simulink model "s_b4a4x32kf_26"  (R2018a)
settings: Solver=VariableStepDiscrete  StartTime=0.0  StopTime=10000  RelTol=1e-3
undefined symbols (not defined in the file): fft_stages, n_bits_ants, n_bits_xengs
libraries: xbsIndex_r4 x21247, casper_library_misc x37, casper_library_scopes x13, casper_library_delays x8, xbsReplacements_r4 x6, xps_library x4
(part 36 of 268)

== system s_b4a4x32kf_26/sys1/xeng_pack_out ==
  note: if we become misaligned,
      | then we must flush the buffers
      | by reading one word, waiting "fifo_latency" clocks,
      | then reading another word until we get rb_done.
  note: the last packet
      | might be shorter!
  note: Delay the output from x-engines,
      | so that only one sends at a time.
  note: we must create a gap
      | between packets from
      | mutliple x-engines to allow
      | the buffers on the output switch
      | ports to drain and NIC card
      | to service the packets.
  data_in : Inport
  valid_in : Inport  Port=2
  pkt_rdy : Inport  Port=3
  rb_done : Inport  Port=4
  timestamp : Inport  Port=5
  xeng_id : Inport  Port=6
  go : Inport  Port=7
  gap_size : Inport  Port=8
  start_offset : Inport  Port=9
  AddSub1 : xbsIndex_r4/AddSub  mode=Subtraction  use_carryin=off  use_carryout=off  en=off  latency=1  precision=User Defined  arith_type=Unsigned  n_bits=vector_bits+1  bin_pt=0  quantization=Truncate  overflow=Saturate  use_behavioral_HDL=on  hw_selection=Fabric  pipelined=off  dbl_ovrd=off  block_type=addsub
      settings: SourceProductName=The database /home/jmanley/.matlab/R2018a/slblocks_master.db is locked, or a table in the database is locked. (database is locked)
  Concat : xbsIndex_r4/Concat  num_inputs=2  dbl_ovrd=off  block_type=concat
      settings: SourceProductName=The database /home/jmanley/.matlab/R2018a/slblocks_master.db is locked, or a table in the database is locked. (database is locked)
  Constant1 : xbsIndex_r4/Constant  const=0  gui_display_data_type=Fixed-point  arith_type=Unsigned  n_bits=spead_lsw  bin_pt=0  preci_type=Single  exp_width=8  frac_width=24  explicit_period=on  period=1  equ=P=C  opselect=C  inp2=PCIN>>17  opr=+  inp1=P  carry=CIN  dbl_ovrd=off  block_type=constant
      settings: SourceProductName=The database /home/jmanley/.matlab/R2018a/slblocks_master.db is locked, or a table in the database is locked. (database is locked)
  Constant15 : xbsIndex_r4/Constant  const=pkt_len  gui_display_data_type=Fixed-point  arith_type=Unsigned  n_bits=vector_bits+1  bin_pt=0  preci_type=Single  exp_width=8  frac_width=24  explicit_period=on  period=1  equ=P=C  opselect=C  inp2=PCIN>>17  opr=+  inp1=P  carry=CIN  dbl_ovrd=off  block_type=constant
      settings: SourceProductName=The database /home/jmanley/.matlab/R2018a/slblocks_master.db is locked, or a table in the database is locked. (database is locked)
  Constant2 : xbsIndex_r4/Constant  const=(vector_len)-1  gui_display_data_type=Fixed-point  arith_type=Unsigned  n_bits=vector_bits+1  bin_pt=0  preci_type=Single  exp_width=8  frac_width=24  explicit_period=on  period=1  equ=P=C  opselect=C  inp2=PCIN>>17  opr=+  inp1=P  carry=CIN  dbl_ovrd=off  block_type=constant
      settings: SourceProductName=The database /home/jmanley/.matlab/R2018a/slblocks_master.db is locked, or a table in the database is locked. (database is locked)
  Constant3 : xbsIndex_r4/Constant  const=vector_len  gui_display_data_type=Fixed-point  arith_type=Unsigned  n_bits=vector_bits+1  bin_pt=0  preci_type=Single  exp_width=8  frac_width=24  explicit_period=on  period=1  equ=P=C  opselect=C  inp2=PCIN>>17  opr=+  inp1=P  carry=CIN  dbl_ovrd=off  block_type=constant
      settings: SourceProductName=The database /home/jmanley/.matlab/R2018a/slblocks_master.db is locked, or a table in the database is locked. (database is locked)
  Constant6 : xbsIndex_r4/Constant  const=heap_len  gui_display_data_type=Fixed-point  arith_type=Unsigned  n_bits=spead_lsw  bin_pt=0  preci_type=Single  exp_width=8  frac_width=24  explicit_period=on  period=1  equ=P=C  opselect=C  inp2=PCIN>>17  opr=+  inp1=P  carry=CIN  dbl_ovrd=off  block_type=constant
      settings: SourceProductName=The database /home/jmanley/.matlab/R2018a/slblocks_master.db is locked, or a table in the database is locked. (database is locked)
  Constant7 : xbsIndex_r4/Constant  const=pkt_len-1  gui_display_data_type=Fixed-point  arith_type=Unsigned  n_bits=pkt_bits  bin_pt=0  preci_type=Single  exp_width=8  frac_width=24  explicit_period=on  period=1  equ=P=C  opselect=C  inp2=PCIN>>17  opr=+  inp1=P  carry=CIN  dbl_ovrd=off  block_type=constant
      settings: SourceProductName=The database /home/jmanley/.matlab/R2018a/slblocks_master.db is locked, or a table in the database is locked. (database is locked)
  Constant8 : xbsIndex_r4/Constant  const=1  gui_display_data_type=Fixed-point  arith_type=Unsigned  n_bits=ceil(log2(fifo_latency))+1  bin_pt=0  preci_type=Single  exp_width=8  frac_width=24  explicit_period=on  period=1  equ=P=C  opselect=C  inp2=PCIN>>17  opr=+  inp1=P  carry=CIN  dbl_ovrd=off  block_type=constant
      settings: SourceProductName=The database /home/jmanley/.matlab/R2018a/slblocks_master.db is locked, or a table in the database is locked. (database is locked)
  Convert{,1..4,6} (6 alike) : xbsIndex_r4/Convert  gui_display_data_type=Fixed-point  arith_type=Unsigned  n_bits=spead_lsw  bin_pt=0  float_type=Single  exp_bits=8  fraction_bits=24  quantization=Truncate  overflow=Wrap  en=off  latency=0  pipeline=off  dbl_ovrd=off  block_type=convert
      settings: SourceProductName=The database /home/jmanley/.matlab/R2018a/slblocks_master.db is locked, or a table in the database is locked. (database is locked)  block_version=11.4
  Counter1 : xbsIndex_r4/Counter  cnt_type=Free Running  cnt_to=1023  operation=Up  start_count=0  cnt_by_val=1  arith_type=Unsigned  n_bits=vector_bits+1  bin_pt=0  load_pin=off  rst=on  en=on  explicit_period=on  period=1  use_behavioral_HDL=off  implementation=Fabric  use_rpm=on  dbl_ovrd=off  block_type=counter
      settings: SourceProductName=The database /home/jmanley/.matlab/R2018a/slblocks_master.db is locked, or a table in the database is locked. (database is locked)  xl_area=[0, 0, 0, 0, 0, 0, 0]
  Delay{,3,10..17,24} (11 alike) : xbsIndex_r4/Delay  rst=off  infoeditControl=Selection of Reset will increase slice count due to use of real FFs and instead of SRLs  en=off  latency=1  reg_retiming=on  dbl_ovrd=off  block_type=delay
      settings: SourceProductName=The database /home/jmanley/.matlab/R2018a/slblocks_master.db is locked, or a table in the database is locked. (database is locked)  block_version=11.4
  Delay1 : xbsIndex_r4/Delay  rst=off  infoeditControl=Selection of Reset will increase slice count due to use of real FFs and instead of SRLs  en=on  latency=1  reg_retiming=on  dbl_ovrd=off  block_type=delay
      settings: SourceProductName=The database /home/jmanley/.matlab/R2018a/slblocks_master.db is locked, or a table in the database is locked. (database is locked)
  Delay2 : xbsIndex_r4/Delay  rst=off  infoeditControl=Selection of Reset will increase slice count due to use of real FFs and instead of SRLs  en=off  latency=fifo_latency  reg_retiming=on  dbl_ovrd=off  block_type=delay
      settings: SourceProductName=The database /home/jmanley/.matlab/R2018a/slblocks_master.db is locked, or a table in the database is locked. (database is locked)  block_version=11.4
  Delay4 : xbsIndex_r4/Delay  rst=off  infoeditControl=Selection of Reset will increase slice count due to use of real FFs and instead of SRLs  en=off  latency=fifo_latency  reg_retiming=on  dbl_ovrd=off  block_type=delay
      settings: SourceProductName=The database /home/jmanley/.matlab/R2018a/slblocks_master.db is locked, or a table in the database is locked. (database is locked)  block_version=11.4
  Delay5 : xbsIndex_r4/Delay  rst=off  infoeditControl=Selection of Reset will increase slice count due to use of real FFs and instead of SRLs  en=on  latency=1  reg_retiming=on  dbl_ovrd=off  block_type=delay
      settings: SourceProductName=The database /home/jmanley/.matlab/R2018a/slblocks_master.db is locked, or a table in the database is locked. (database is locked)
  Delay7 : xbsIndex_r4/Delay  rst=on  infoeditControl=Selection of Reset will increase slice count due to use of real FFs and instead of SRLs  en=on  latency=1  reg_retiming=on  dbl_ovrd=off  block_type=delay
      settings: SourceProductName=The database /home/jmanley/.matlab/R2018a/slblocks_master.db is locked, or a table in the database is locked. (database is locked)
  Delay8 : xbsIndex_r4/Delay  rst=on  infoeditControl=Selection of Reset will increase slice count due to use of real FFs and instead of SRLs  en=on  latency=1  reg_retiming=on  dbl_ovrd=off  block_type=delay
      settings: SourceProductName=The database /home/jmanley/.matlab/R2018a/slblocks_master.db is locked, or a table in the database is locked. (database is locked)
  Delay9 : xbsIndex_r4/Delay  rst=on  infoeditControl=Selection of Reset will increase slice count due to use of real FFs and instead of SRLs  en=on  latency=1  reg_retiming=on  dbl_ovrd=off  block_type=delay
      settings: SourceProductName=The database /home/jmanley/.matlab/R2018a/slblocks_master.db is locked, or a table in the database is locked. (database is locked)
  Inverter{1..3,6..7} (5 alike) : xbsIndex_r4/Inverter  en=off  latency=0  dbl_ovrd=off  block_type=inv
      settings: SourceProductName=The database /home/jmanley/.matlab/R2018a/slblocks_master.db is locked, or a table in the database is locked. (database is locked)  block_version=11.4
  Logical{1,3..5,13..14} (6 alike) : xbsIndex_r4/Logical  logical_function=OR  inputs=2  en=off  latency=0  precision=Full  arith_type=Unsigned  n_bits=8  bin_pt=2  align_bp=on  dbl_ovrd=off  block_type=logical
      settings: SourceProductName=The database /home/jmanley/.matlab/R2018a/slblocks_master.db is locked, or a table in the database is locked. (database is locked)  xl_area=[0, 0, 0, 0, 0, 0, 0]
  Logical{2,8..12,15} (7 alike) : xbsIndex_r4/Logical  logical_function=AND  inputs=2  en=off  latency=0  precision=Full  arith_type=Unsigned  n_bits=8  bin_pt=2  align_bp=on  dbl_ovrd=off  block_type=logical
      settings: SourceProductName=The database /home/jmanley/.matlab/R2018a/slblocks_master.db is locked, or a table in the database is locked. (database is locked)  xl_area=[0, 0, 0, 0, 0, 0, 0]
  Logical17 : xbsIndex_r4/Logical  logical_function=AND  inputs=2  en=off  latency=1  precision=Full  arith_type=Unsigned  n_bits=8  bin_pt=2  align_bp=on  dbl_ovrd=off  block_type=logical
      settings: SourceProductName=The database /home/jmanley/.matlab/R2018a/slblocks_master.db is locked, or a table in the database is locked. (database is locked)  xl_area=[0, 0, 0, 0, 0, 0, 0]
  Logical18 : xbsIndex_r4/Logical  logical_function=AND  inputs=2  en=off  latency=1  precision=Full  arith_type=Unsigned  n_bits=8  bin_pt=2  align_bp=on  dbl_ovrd=off  block_type=logical
      settings: SourceProductName=The database /home/jmanley/.matlab/R2018a/slblocks_master.db is locked, or a table in the database is locked. (database is locked)  xl_area=[0, 0, 0, 0, 0, 0, 0]
  Logical19 : xbsIndex_r4/Logical  logical_function=AND  inputs=2  en=off  latency=1  precision=Full  arith_type=Unsigned  n_bits=8  bin_pt=2  align_bp=on  dbl_ovrd=off  block_type=logical
      settings: SourceProductName=The database /home/jmanley/.matlab/R2018a/slblocks_master.db is locked, or a table in the database is locked. (database is locked)  xl_area=[0, 0, 0, 0, 0, 0, 0]
  Logical7 : xbsIndex_r4/Logical  logical_function=XOR  inputs=2  en=off  latency=0  precision=Full  arith_type=Unsigned  n_bits=8  bin_pt=2  align_bp=on  dbl_ovrd=off  block_type=logical
      settings: SourceProductName=The database /home/jmanley/.matlab/R2018a/slblocks_master.db is locked, or a table in the database is locked. (database is locked)  xl_area=[0, 0, 0, 0, 0, 0, 0]
  Mux1 : xbsIndex_r4/Mux  inputs=2  en=off  latency=1  precision=Full  arith_type="Signed  (2's comp)"  n_bits=8  bin_pt=2  quantization=Truncate  overflow=Wrap  dbl_ovrd=off  block_type=mux
      settings: SourceProductName=The database /home/jmanley/.matlab/R2018a/slblocks_master.db is locked, or a table in the database is locked. (database is locked)  xl_area=[0, 0, 0, 0, 0, 0, 0]
  Reinterpret : xbsIndex_r4/Reinterpret  force_arith_type=on  arith_type=Unsigned  force_bin_pt=on  bin_pt=0  block_type=reinterpret
      settings: SourceProductName=The database /home/jmanley/.matlab/R2018a/slblocks_master.db is locked, or a table in the database is locked. (database is locked)  infoedit="Changes signal type without altering the binary representation.   You can changed the signal between signed and unsigned, and relocate the binary point.<br><br>Hardware notes: In hardware this block costs nothing.<br><br>Example:  Suppose the input is 6 bits wide, signed, with 2 fractional bits, and the output is forced to unsigned with 0 fractional bits.  Then an input of -2.0 (1110.00 in binary 2's complement) becomes an output of 56 (111000 in binary)."
  Relational1 : xbsIndex_r4/Relational  mode=a=b  op_type=Bool  en=off  latency=0  dbl_ovrd=off  block_type=relational
      settings: SourceProductName=The database /home/jmanley/.matlab/R2018a/slblocks_master.db is locked, or a table in the database is locked. (database is locked)  xl_area=[0, 0, 0, 0, 0, 0, 0]  block_version=10.1.3
  Relational2 : xbsIndex_r4/Relational  mode=a<b  op_type=Bool  en=off  latency=0  dbl_ovrd=off  block_type=relational
      settings: SourceProductName=The database /home/jmanley/.matlab/R2018a/slblocks_master.db is locked, or a table in the database is locked. (database is locked)  xl_area=[0, 0, 0, 0, 0, 0, 0]  block_version=10.1.3
  Relational4 : xbsIndex_r4/Relational  mode=a=b  op_type=Bool  en=off  latency=0  dbl_ovrd=off  block_type=relational
      settings: SourceProductName=The database /home/jmanley/.matlab/R2018a/slblocks_master.db is locked, or a table in the database is locked. (database is locked)  xl_area=[0, 0, 0, 0, 0, 0, 0]  block_version=10.1.3
  Relational5 : xbsIndex_r4/Relational  mode=a=b  op_type=Bool  en=off  latency=0  dbl_ovrd=off  block_type=relational
      settings: SourceProductName=The database /home/jmanley/.matlab/R2018a/slblocks_master.db is locked, or a table in the database is locked. (database is locked)  xl_area=[0, 0, 0, 0, 0, 0, 0]  block_version=10.1.3
  Shift1 : xbsIndex_r4/Shift  shift_dir=Left  shift_bits=n_bits_word_size  en=off  latency=0  precision=Full  arith_type="Signed  (2's comp)"  n_bits=16  bin_pt=14  quantization=Truncate  overflow=Wrap  dbl_ovrd=off  block_type=shift
      settings: SourceProductName=The database /home/jmanley/.matlab/R2018a/slblocks_master.db is locked, or a table in the database is locked. (database is locked)
  Shift2 : xbsIndex_r4/Shift  shift_dir=Left  shift_bits=n_bits_chans  en=off  latency=0  precision=Full  arith_type="Signed  (2's comp)"  n_bits=16  bin_pt=14  quantization=Truncate  overflow=Wrap  dbl_ovrd=off  block_type=shift
      settings: SourceProductName=The database /home/jmanley/.matlab/R2018a/slblocks_master.db is locked, or a table in the database is locked. (database is locked)
  Slice : xbsIndex_r4/Slice  nbits=pkt_bits  boolean_output=off  mode=Lower Bit Location + Width  bit1=0  base1=MSB of Input  bit0=0  base0=LSB of Input  dbl_ovrd=off  block_type=slice
      settings: SourceProductName=The database /home/jmanley/.matlab/R2018a/slblocks_master.db is locked, or a table in the database is locked. (database is locked)
  Slice1 : xbsIndex_r4/Slice  nbits=1  boolean_output=off  mode=Two Bit Locations  bit1=0  base1=MSB of Input  bit0=n_bits_timestamp_padding  base0=LSB of Input  dbl_ovrd=off  block_type=slice
      settings: SourceProductName=The database /home/jmanley/.matlab/R2018a/slblocks_master.db is locked, or a table in the database is locked. (database is locked)
  edge_detect : Subsystem  AncestorBlock=casper_library_misc/edge_detect  mask(edge_detect){edge=Rising, polarity=Active High, x_in=[0 0.08 0.08 0.16 0.16 0.24 0.24 0.32 0.32 0.4], y_in=[-1 -1  1  1  1  1  1  1  1  1], x_out=[0.6 0.68 0.68 0.76 0.76 0.84 0.84 0.92 0.92 1], y_out=[-1 -1  1  1 -1 -1 -1 -1 -1 -1]}
      mask prompts: edge "Edge Type"; polarity "Output Polarity"; x_in "Input X Positions"; y_in "Input Y Positions"; x_out "Output X Positions"; y_out "Output Y Positions"
      mask help: Output is active for one-cycle after each edge of the specified type (i.e. rising, falling or both).
      mask init: same as s_b4a4x32kf_26/edge_detect
      settings: AttributesFormatString=|
      | rising edges
      | active high
      mask Help: Output is active for one-cycle after each edge of the specified type (i.e. rising, falling, or both).  Latency is zero.
      mask TypeOptions edge: Rising | Falling | Both
      mask TypeOptions polarity: Active High | Active Low
      mask Display:
      | plot(x_in_num,0.5+y_in_num*0.2);
      | plot(x_out_num,0.5+y_out_num*0.2);
  edge_detect1 : Subsystem  AncestorBlock=casper_library_misc/edge_detect  mask(edge_detect){edge=Rising, polarity=Active High, x_in=[0 0.08 0.08 0.16 0.16 0.24 0.24 0.32 0.32 0.4], y_in=[-1 -1  1  1  1  1  1  1  1  1], x_out=[0.6 0.68 0.68 0.76 0.76 0.84 0.84 0.92 0.92 1], y_out=[-1 -1  1  1 -1 -1 -1 -1 -1 -1]}
      mask prompts: edge "Edge Type"; polarity "Output Polarity"; x_in "Input X Positions"; y_in "Input Y Positions"; x_out "Output X Positions"; y_out "Output Y Positions"
      mask help: Output is active for one-cycle after each edge of the specified type (i.e. rising, falling or both).
      mask init: same as s_b4a4x32kf_26/edge_detect
      settings: AttributesFormatString=|
      | rising edges
      | active high
      mask Help: Output is active for one-cycle after each edge of the specified type (i.e. rising, falling, or both).  Latency is zero.
      mask TypeOptions edge: Rising | Falling | Both
      mask TypeOptions polarity: Active High | Active Low
      mask Display:
      | plot(x_in_num,0.5+y_in_num*0.2);
      | plot(x_out_num,0.5+y_out_num*0.2);
  edge_detect2 : Subsystem  AncestorBlock=casper_library_misc/edge_detect  mask(edge_detect){edge=Rising, polarity=Active High, x_in=[0 0.08 0.08 0.16 0.16 0.24 0.24 0.32 0.32 0.4], y_in=[-1 -1  1  1  1  1  1  1  1  1], x_out=[0.6 0.68 0.68 0.76 0.76 0.84 0.84 0.92 0.92 1], y_out=[-1 -1  1  1 -1 -1 -1 -1 -1 -1]}
      mask prompts: edge "Edge Type"; polarity "Output Polarity"; x_in "Input X Positions"; y_in "Input Y Positions"; x_out "Output X Positions"; y_out "Output Y Positions"
      mask help: Output is active for one-cycle after each edge of the specified type (i.e. rising, falling or both).
      mask init: same as s_b4a4x32kf_26/edge_detect
      settings: AttributesFormatString=|
      | rising edges
      | active high
      mask Help: Output is active for one-cycle after each edge of the specified type (i.e. rising, falling, or both).  Latency is zero.
      mask TypeOptions edge: Rising | Falling | Both
      mask TypeOptions polarity: Active High | Active Low
      mask Display:
      | plot(x_in_num,0.5+y_in_num*0.2);
      | plot(x_out_num,0.5+y_out_num*0.2);
  edge_detect3 : Subsystem  AncestorBlock=casper_library_misc/edge_detect  mask(edge_detect){edge=Rising, polarity=Active High, x_in=[0 0.08 0.08 0.16 0.16 0.24 0.24 0.32 0.32 0.4], y_in=[-1 -1  1  1  1  1  1  1  1  1], x_out=[0.6 0.68 0.68 0.76 0.76 0.84 0.84 0.92 0.92 1], y_out=[-1 -1  1  1 -1 -1 -1 -1 -1 -1]}
      mask prompts: edge "Edge Type"; polarity "Output Polarity"; x_in "Input X Positions"; y_in "Input Y Positions"; x_out "Output X Positions"; y_out "Output Y Positions"
      mask help: Output is active for one-cycle after each edge of the specified type (i.e. rising, falling or both).
      mask init: same as s_b4a4x32kf_26/edge_detect
      settings: AttributesFormatString=|
      | rising edges
      | active high
      mask Help: Output is active for one-cycle after each edge of the specified type (i.e. rising, falling, or both).  Latency is zero.
      mask TypeOptions edge: Rising | Falling | Both
      mask TypeOptions polarity: Active High | Active Low
      mask Display:
      | plot(x_in_num,0.5+y_in_num*0.2);
      | plot(x_out_num,0.5+y_out_num*0.2);
  edge_detect7 : Subsystem  mask(edge_detect){edge=Rising, polarity=Active High, x_in=[0 0.08 0.08 0.16 0.16 0.24 0.24 0.32 0.32 0.4], y_in=[-1 -1  1  1  1  1  1  1  1  1], x_out=[0.6 0.68 0.68 0.76 0.76 0.84 0.84 0.92 0.92 1], y_out=[-1 -1  1  1 -1 -1 -1 -1 -1 -1]}
      mask prompts: edge "Edge Type"; polarity "Output Polarity"; x_in "Input X Positions"; y_in "Input Y Positions"; x_out "Output X Positions"; y_out "Output Y Positions"
      mask help: Output is active for one-cycle after each edge of the specified type (i.e. rising, falling or both).
      mask init: same as s_b4a4x32kf_26/edge_detect
      settings: AttributesFormatString=|
      | rising edges
      | active high
      mask Help: Output is active for one-cycle after each edge of the specified type (i.e. rising, falling, or both).  Latency is zero.
      mask TypeOptions edge: Rising | Falling | Both
      mask TypeOptions polarity: Active High | Active Low
      mask Display:
      | plot(x_in_num,0.5+y_in_num*0.2);
      | plot(x_out_num,0.5+y_out_num*0.2);
  gap_creator2 : xbsIndex_r4/Counter  cnt_type=Free Running  cnt_to=Inf  operation=Up  start_count=0  cnt_by_val=1  arith_type=Unsigned  n_bits=n_bits_max_gap  bin_pt=0  load_pin=off  rst=on  en=on  explicit_period=on  period=1  use_behavioral_HDL=off  implementation=Fabric  dbl_ovrd=off  block_type=counter
      settings: SourceProductName=The database /home/jmanley/.matlab/R2018a/slblocks_master.db is locked, or a table in the database is locked. (database is locked)
  gap_creator4 : xbsIndex_r4/Counter  cnt_type=Free Running  cnt_to=Inf  operation=Up  start_count=0  cnt_by_val=1  arith_type=Unsigned  n_bits=n_bits_max_gap  bin_pt=0  load_pin=off  rst=on  en=on  explicit_period=on  period=1  use_behavioral_HDL=off  implementation=Fabric  dbl_ovrd=off  block_type=counter
      settings: SourceProductName=The database /home/jmanley/.matlab/R2018a/slblocks_master.db is locked, or a table in the database is locked. (database is locked)
  gap_done2 : xbsIndex_r4/Relational  mode=a<b  op_type=Bool  en=off  latency=1  dbl_ovrd=off  block_type=relational
      settings: SourceProductName=The database /home/jmanley/.matlab/R2018a/slblocks_master.db is locked, or a table in the database is locked. (database is locked)
  gap_done4 : xbsIndex_r4/Relational  mode=a>b  op_type=Bool  en=off  latency=1  dbl_ovrd=off  block_type=relational
      settings: SourceProductName=The database /home/jmanley/.matlab/R2018a/slblocks_master.db is locked, or a table in the database is locked. (database is locked)
  pack_xeng : Subsystem  Tag=casper:spead_pack  AncestorBlock=casper_library_communications/spead_pack  mask(pkt_pack_mask){max_pkt_len_bits=8, header_ids=0x1600, 0x4103, header_ind_ids=0x1800, spead_msw=64, spead_lsw=48, spead_version=4, bytes_per_word=8}
      mask prompts: max_pkt_len_bits "Max pkt length, 2^? 64-bit words"; header_ids "SPEAD direct address IDs (decimal)"; header_ind_ids "SPEAD indirect address IDs (decimal)"; spead_msw "SPEAD Flavour (MSw)"; spead_lsw "SPEAD Flavour (LSw)"; spead_version "SPEAD version"; bytes_per_word "Word size, in bytes"
      mask help:
      | This block generates SPEAD-compliant packets from a datastream.
      |
      | Packets are created with a fixed header followed by a number of 64-bit items.
      |
      | Requires a 64-bit data stream.
      |
      | The data_ready signal is one cycle BEFORE valid data! Does not have to be with a valid signal either.
      mask init:
      | % if floor(log2(bytes_per_word)) ~= log2(bytes_per_word)
      | %     error('Bytes per word should be a power of two.');
      | % end
      | % 
      | % spead_pack_init(gcb)
  payload_cnt4 : xbsIndex_r4/Counter  cnt_type=Count Limited  cnt_to=max((fifo_latency + 1),2)  operation=Up  start_count=0  cnt_by_val=1  arith_type=Unsigned  n_bits=ceil(log2(fifo_latency))+1  bin_pt=0  load_pin=off  rst=on  en=on  explicit_period=on  period=1  use_behavioral_HDL=off  implementation=Fabric  use_rpm=on  dbl_ovrd=off  block_type=counter
      settings: SourceProductName=The database /home/jmanley/.matlab/R2018a/slblocks_master.db is locked, or a table in the database is locked. (database is locked)  xl_area=[0, 0, 0, 0, 0, 0, 0]
  status : Subsystem  Tag=xps:sw_reg  AncestorBlock=xps_library/software register  mask(swreg){io_dir=To Processor, io_delay=1, sample_period=1, names=[pkt_cnt align_err_cnt overflow_err_cnt], bitwidths=[16 8 8], bin_pts=0, arith_types=0, sim_port=off, show_format=off}
      mask prompts: io_dir "I/O direction"; io_delay "I/O delay"; sample_period "Sample period"; names "Bitfield names [msb...lsb]"; bitwidths "Bitfield widths"; bin_pts "Bitfield binary pts"; arith_types "Bitfield types, ufix=0, fix=1, bool=2"; sim_port "Provide sim input/output?"; show_format "Print format string?"
      mask help: A 32-bit software-accessible register. Can be divided into bitfields of varying widths and types using the fields in the block mask.
      mask init:
      | try
      |     swreg_init(gcb)
      | catch ex
      |     disp(sprintf('%s: %s', gcb, ex.message))
      |     errordlg(ex.message)
      | end
      settings: AttributesFormatString=3 outputs
      mask TypeOptions io_dir: To Processor | From Processor
      mask Callback io_dir:
      | mask_enables = get_param(gcb, 'MaskEnables');
      | mask_names = get_param(gcb, 'MaskNames');
      | if strcmp(get_param(gcb, 'io_dir'), 'To Processor'),
      |     mask_enables{ismember(mask_names, 'sample_period')} = 'off';
      | else
      |     mask_enables{ismember(mask_names, 'sample_period')} = 'on';
      | end
      | set_param(gcb, 'MaskEnables', mask_enables);
  vacc_monitor3 : Subsystem
  data_out : Outport
  valid_out : Outport  Port=2
  eof : Outport  Port=3
  err : Outport  Port=4
  fetch : Outport  Port=5
  pkt_ready : Outport  Port=6
  wires:
  Convert6/1 -> Shift2/1
  Constant1/1 -> pack_xeng/10(hdr8_0x1800)
  Convert2/1 -> [heap_cnt]
  Concat/1 -> Convert2/1
  [xeng_id] -> Concat/2
  Slice1/1 -> Concat/1
  [timestamp] -> Slice1/1
  gap_size/1 -> [gap_size]
  Delay13/1 -> pack_xeng/9(hdr6_0x4103_DIR)
  [freq_offset] -> Delay13/1
  Shift2/1 -> [freq_offset]
  [xeng_id] -> Convert6/1
  Convert4/1 -> Delay16/1
  pack_xeng/3(eof) -> Logical3/1
  Logical3/1 -> [eof_out], eof/1
  [end_of_vector] -> Logical5/1
  Logical5/1 -> [eof]
  Logical2/1 -> [rb_done]
  xeng_id/1 -> [xeng_id]
  Reinterpret/1 -> [data_input]
  Slice/1 -> Relational1/1
  Counter1/1 -> [vector_position], Slice/1, Relational5/1
  timestamp/1 -> Delay5/1
  Delay5/1 -> [timestamp]
  [vector_start] -> Delay5/2
  Constant2/1 -> Relational5/2
  Relational5/1 -> [end_of_vector]
  data_in/1 -> Reinterpret/1, [raw_data_input]
  valid_in/1 -> Logical2/1, [valid_input]
  pkt_rdy/1 -> [pkt_rdy]
  rb_done/1 -> Logical2/2
  [valid_input] -> [valid_output]
  [fetch_pld] -> Counter1/2
  [vector_start] -> Counter1/1
  Constant7/1 -> Relational1/2
  Relational1/1 -> Logical5/2
  pack_xeng/1(data_out) -> data_out/1, [data_out]
  [vector_position] -> Delay1/1
  Delay1/1 -> AddSub1/2, Delay17/1
  [get_a_pkt] -> Delay1/2
  [rb_done] -> Logical7/1
  [end_of_vector] -> Delay2/1
  Delay17/1 -> Convert/1
  Convert/1 -> Shift1/1
  [vector_start] -> Logical4/1
  Logical4/1 -> Delay4/1
  [go] -> Logical8/1
  Logical8/1 -> Delay3/1
  Delay7/1 -> [busy], edge_detect/1(in)
  edge_detect/1(out) -> [vector_start]
  Inverter2/1 -> Logical10/1
  Logical10/1 -> Delay7/1, Delay7/3
  [end_of_vector] -> Logical1/2
  [go] -> Delay/1
  edge_detect1/1(out) -> Logical10/2
  [busy] -> Inverter2/1
  Delay/1 -> edge_detect1/1(in)
  Delay2/1 -> Logical7/2
  [get_a_pkt] -> Inverter1/1
  Delay3/1 -> Logical4/2
  Delay4/1 -> Delay8/1, Delay8/3
  edge_detect2/1(out) -> [get_a_pkt]
  Delay8/1 -> [busy_pkt], edge_detect2/1(in)
  [eof] -> Delay8/2
  [busy] -> Logical8/2
  Inverter1/1 -> Logical9/1
  Logical9/1 -> [fetch_pld]
  Logical7/1 -> Delay9/1, Delay9/3, [err]
  [rb_done] -> Logical12/2
  payload_cnt4/1 -> Relational4/2
  Constant8/1 -> Relational4/1
  Delay9/1 -> payload_cnt4/2, [flushing]
  Relational4/1 -> [stutter_flush]
  Logical1/1 -> Delay7/2
  [err] -> Logical1/1
  [valid_output] -> Logical11/1
  Inverter3/1 -> Logical11/2, Logical15/2
  [flushing] -> Inverter3/1
  Logical12/1 -> Delay9/2, payload_cnt4/1
  [flushing] -> Logical12/1
  Logical13/1 -> fetch/1
  [fetch_pld] -> Logical13/1
  [stutter_flush] -> Logical13/2
  Constant15/1 -> Relational2/2, Mux1/2
  Mux1/1 -> Convert1/1
  Relational2/1 -> Mux1/1
  Constant3/1 -> AddSub1/1
  AddSub1/1 -> Mux1/3, Relational2/1
  Convert1/1 -> [pld_len]
  Shift1/1 -> [heap_offset]
  go/1 -> [go]
  [data_input] -> Delay11/1
  [heap_cnt] -> Convert3/1
  [heap_offset] -> Delay14/1
  Logical11/1 -> Delay10/1
  pack_xeng/2(valid_out) -> valid_out/1
  [pld_len] -> Delay15/1
  Logical14/1 -> Logical3/2, err/1
  pack_xeng/4(data_overflow) -> [data_overflow], Logical14/2
  [err] -> Logical14/1
  [valid_output] -> Logical15/1
  edge_detect3/1(out) -> pack_xeng/1(data256_ready)
  Logical15/1 -> edge_detect3/1(in)
  Delay10/1 -> pack_xeng/2(data256_valid)
  Delay11/1 -> pack_xeng/3(data256)
  Delay12/1 -> pack_xeng/4(hdr_heap_id)
  Constant6/1 -> pack_xeng/5(hdr_heap_size)
  Delay14/1 -> pack_xeng/6(hdr_heap_offset)
  Delay15/1 -> pack_xeng/7(hdr_pkt_len_words)
  Delay16/1 -> pack_xeng/8(hdr5_0x1600_DIR)
  [busy_pkt] -> Logical9/2
  Convert3/1 -> Delay12/1
  [timestamp] -> Convert4/1
  start_offset/1 -> [start_offset]
  [cnt_rst] -> vacc_monitor3/1(cnt_rst)
  vacc_monitor3/1(pkt_cnt) -> status/1(out_pkt_cnt)
  [eof_out] -> vacc_monitor3/2(eof)
  [err] -> vacc_monitor3/3(error)
  [data_overflow] -> vacc_monitor3/4(overflow)
  vacc_monitor3/2(error_cnt) -> status/2(out_align_err_cnt)
  vacc_monitor3/3(overflow_cnt) -> status/3(out_overflow_err_cnt)
  Inverter7/1 -> Logical18/1
  gap_creator2/1 -> gap_done2/1, [gap_count]
  gap_done2/1 -> gap_creator2/2, Inverter7/1
  [eof] -> Delay24/1
  [start_offset] -> gap_done4/2
  Logical17/1 -> pkt_ready/1
  [gap_size] -> gap_done2/2
  gap_done4/1 -> Inverter6/1, Logical17/2
  [pkt_rdy] -> Logical18/2
  [rb_done] -> gap_creator4/1
  Logical19/1 -> gap_creator4/2
  edge_detect7/1(out) -> gap_creator2/1
  Inverter6/1 -> Logical19/2
  gap_creator4/1 -> gap_done4/1
  Delay24/1 -> edge_detect7/1(in)
  Logical18/1 -> Logical19/1, Logical17/1
